simulink model "Rotary_inverted_pendulum_simscape_model"  (R2026b)
settings: Solver=VariableStepAuto  StopTime=10  EnableMultiTasking=on
InitFcn:
  | Rotary_inverted_pendulum_params;
values from neighbouring files (symbols this model uses):
  A = [0 0 1.58599833727e-11 -4.90689813272e-13 0 0 11.773740367 153.017565535 1 0 -0.668730280726 -0.988272810616 ... (16 elements, 4x4)]    [Rotary_inverted_pendulum_control_.mat]    (also in Rotary_inverted_pendulum_params.m = A_hand; Rotary_inverted_pendulum_symbolic.m = zeros(4,4))
  alpha_0 = 170    [Rotary_inverted_pendulum_params.m]
  alpha_cal = -3.678    [Rotary_inverted_pendulum_params.m]
  B = [0 0 3.48321726757 5.14775001613]    [Rotary_inverted_pendulum_control_.mat]    (also in Rotary_inverted_pendulum_params.m = B_hand; Rotary_inverted_pendulum_symbolic.m = zeros(4,1))
  C = [1 0 0 0; 0 1 0 0]    [Rotary_inverted_pendulum_params.m]
  D = [0; 0]    [Rotary_inverted_pendulum_params.m]
  K_c = place(A,B,[-8 -5 -6 -1])    [Rotary_inverted_pendulum_params.m]
  km = 0.035    [Rotary_inverted_pendulum_params.m]
  kt = 0.035    [Rotary_inverted_pendulum_params.m]
  L = 264e-6    (= 0.000264)    [Rotary_inverted_pendulum_params.m]
  L_o = place(A',C',5*[-8 -5 -6 -1])'    [Rotary_inverted_pendulum_params.m]
  link_mass = 0.08    [Rotary_inverted_pendulum_params.m]
  N = 1    [Rotary_inverted_pendulum_params.m]
  p_mass = 0.1    [Rotary_inverted_pendulum_params.m]
  R = 7.14    [Rotary_inverted_pendulum_params.m]    (also in Rotary_inverted_pendulum_symbolic.m = 2)
  rod_mass = 0.05    [Rotary_inverted_pendulum_params.m]
  rt1 = 7/2    (= 3.5)    [Rotary_inverted_pendulum_params.m]
  rt2 = 8.5-0.4    (= 8.1)    [Rotary_inverted_pendulum_params.m]
  V_max = 24    [Rotary_inverted_pendulum_params.m]
undefined symbols (not defined in the file or in its folder): K, L_q, X, Y, Z
libraries: sm_lib x123, nesl_utility x29, simulink x10
(part 4 of 4)

== system Rotary_inverted_pendulum_simscape_model/Inverted Pendulum System6/Physical Model/Pendulum (Link 3) ==
  Pendulum (Link 3) : sm_lib/Body Elements/File Solid  ExtGeomFileName=C:\Users\Mrsh\Downloads\Pedulum(1).STEP  UnitType=FromFile  ExtGeomFileUnits=cm  StepReaderType=HEX  ExportConvexHullGeometry=off  InertiaType=CalculateFromGeometry  BasedOnType=Mass  Density=1000  DensityUnits=kg/m^3  Mass=p_mass  MassUnits=kg  CenterOfMass=[0 0 0]  CenterOfMassUnits=m  MomentsOfInertia=[1 1 1]  MomentsOfInertiaUnits=kg*m^2  ProductsOfInertia=[0 0 0]  ProductsOfInertiaUnits=kg*m^2  GraphicType=FromGeometry  MarkerShape=Sphere  MarkerSize=10  GraphicVisPropType=AdvancedVisualProperties  GraphicDiffuseColor=[0.6902 0.6902 0.6902]  GraphicOpacity=1.0  GraphicSpecularColor=[0.549 0.549 0.549]  GraphicAmbientColor=[0.15 0.15 0.15 1.0]  GraphicEmissiveColor=[0.0 0.0 0.0 1.0]  GraphicShininess=75  DoExposeReferenceFrame=off  SerializedFrames=<Frames><Frame><Id>Frame1</Id><Value><Name>F1</Name><Origin><Source>GeometricFeature</Source><FeatureName>planar surface 53</FeatureName></Origin><PrimaryAxis><DefinedDirection>-Y</DefinedDirection><Source>ReferenceFrame</Source><SourceDirection>+Z</SourceDirection><FeatureName></FeatureName></PrimaryAxis><SecondaryAxis><DefinedDirection>+X</DefinedDirection><Source>ReferenceFrame</Source><SourceDirection>+X</SourceDirection><FeatureName></FeatureName></SecondaryAxis></Value></Frame></Frames>
  Pendulum Angle : sm_lib/Frames and Transforms/Rigid Transform  RotationMethod=StandardAxis  FollAlignAxisA=+X  BaseAlignAxisA=+Y  FollAlignAxisB=+Y  BaseAlignAxisB=+Z  RotationStandardAxis=+Z  RotationAngle=alpha_0-180+alpha_cal  RotationAngleUnits=deg  RotationArbitraryAxis=[0 0 1]  RotationSequenceAxes=FollowerAxes  RotationSequence=XYX  RotationSequenceAngles=[0 0 0]  RotationSequenceAnglesUnits=deg  RotationMatrix=[1 0 0; 0 1 0; 0 0 1]  Quaternion=[1 0 0 0]  TranslationMethod=None  TranslationCartesianOffset=0  TranslationCartesianOffsetUnits=cm  TranslationStandardAxis=+Z  TranslationStandardOffset=0  TranslationStandardOffsetUnits=cm  TranslationROffset=0  TranslationROffsetUnits=m  TranslationThetaOffset=0  TranslationThetaOffsetUnits=deg  TranslationZOffset=0  TranslationZOffsetUnits=m
  Rigid Transform1 : sm_lib/Frames and Transforms/Rigid Transform  RotationMethod=StandardAxis  FollAlignAxisA=+X  BaseAlignAxisA=+Y  FollAlignAxisB=+Y  BaseAlignAxisB=+Z  RotationStandardAxis=+Y  RotationAngle=180  RotationAngleUnits=deg  RotationArbitraryAxis=[0 0 1]  RotationSequenceAxes=FollowerAxes  RotationSequence=XYX  RotationSequenceAngles=[0 0 0]  RotationSequenceAnglesUnits=deg  RotationMatrix=[1 0 0; 0 1 0; 0 0 1]  Quaternion=[1 0 0 0]  TranslationMethod=Cartesian  TranslationCartesianOffset=[0 0 3]  TranslationCartesianOffsetUnits=cm  TranslationStandardAxis=+Z  TranslationStandardOffset=0  TranslationStandardOffsetUnits=cm  TranslationROffset=0  TranslationROffsetUnits=m  TranslationThetaOffset=0  TranslationThetaOffsetUnits=deg  TranslationZOffset=0  TranslationZOffsetUnits=m
  Conn1 : PMIOPort  Side=Left
  connections:
  Conn1/RConn1 -- Pendulum Angle/LConn1
  Rigid Transform1/LConn1 -- Pendulum Angle/RConn1
  Rigid Transform1/RConn1 -- Pendulum (Link 3)/LConn1
